simulink model "untitled1"  (R2023b)
settings: Solver=VariableStepAuto  StartTime=0.0  StopTime=20  RelTol=1e-3
settings Model: Creator=user  LastModifiedBy=user

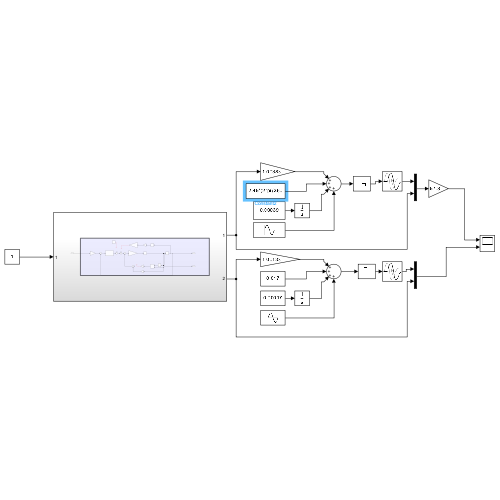
[thumbnail: Simulink's stored preview of the top-level diagram]
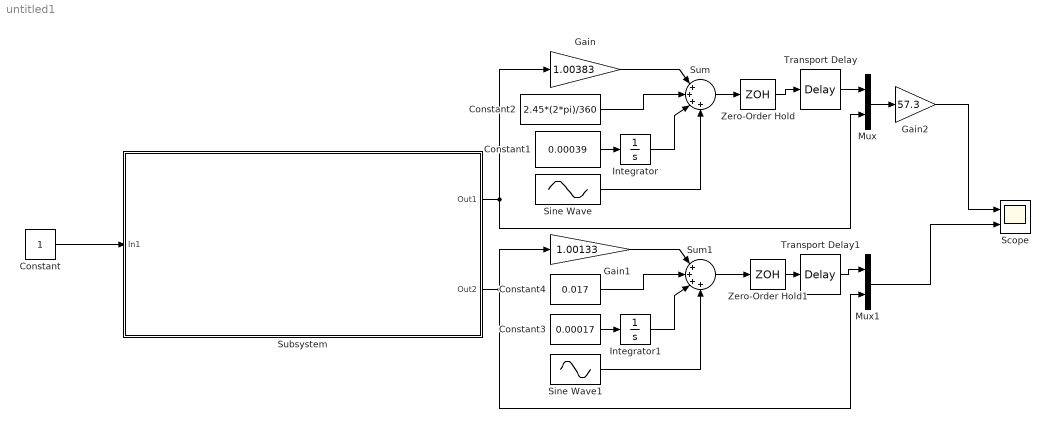
== system untitled1 ==
  Constant : Constant
  Constant1 : Constant  Value=0.00039
  Constant2 : Constant  Value=2.45*(2*pi)/360
  Constant3 : Constant  Value=0.00017
  Constant4 : Constant  Value=0.017
  Gain : Gain  Gain=1.00383
  Gain1 : Gain  Gain=1.00133
  Gain2 : Gain  Gain=57.3
  Integrator : Integrator
  Integrator1 : Integrator
  Mux : Mux  Inputs=2
  Mux1 : Mux  Inputs=2
  Scope : Scope  NumInputPorts=2
  Sine Wave : Sin  Amplitude=0.003  Frequency=50  SampleTime=0
  Sine Wave1 : Sin  Amplitude=0.00017  Frequency=25  SampleTime=0
  Subsystem : Subsystem
  Sum : Sum  Inputs=|++++
  Sum1 : Sum  Inputs=|++++
  Transport Delay : TransportDelay  DelayTime=0.002
  Transport Delay1 : TransportDelay  DelayTime=0.002
  Zero-Order Hold : ZeroOrderHold  SampleTime=0.1
  Zero-Order Hold1 : ZeroOrderHold  SampleTime=0.1
  wires:
  Constant/1 -> Subsystem/1(In1)
  Sum/1 -> Zero-Order Hold/1
  Constant1/1 -> Integrator/1
  Subsystem/1(Out1) -> Gain/1, Mux/2
  Gain/1 -> Sum/1
  Constant2/1 -> Sum/2
  Integrator/1 -> Sum/3
  Sine Wave/1 -> Sum/4
  Zero-Order Hold/1 -> Transport Delay/1
  Transport Delay1/1 -> Mux1/1
  Gain1/1 -> Sum1/1
  Zero-Order Hold1/1 -> Transport Delay1/1
  Integrator1/1 -> Sum1/3
  Sine Wave1/1 -> Sum1/4
  Subsystem/2(Out2) -> Gain1/1, Mux1/2
  Constant4/1 -> Sum1/2
  Sum1/1 -> Zero-Order Hold1/1
  Constant3/1 -> Integrator1/1
  Mux/1 -> Gain2/1
  Mux1/1 -> Scope/2
  Gain2/1 -> Scope/1
  Transport Delay/1 -> Mux/1

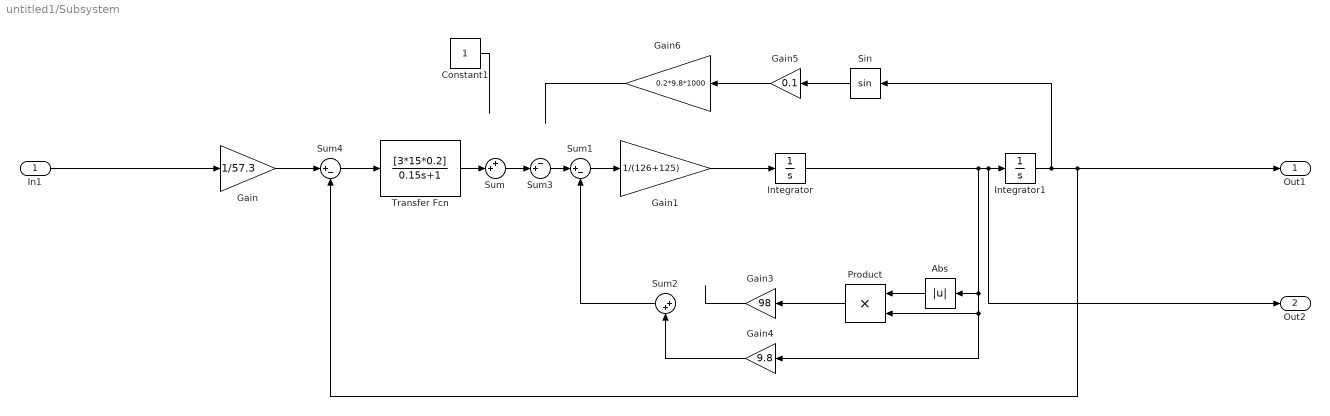
== system untitled1/Subsystem ==
  In1 : Inport
  Abs : Abs  SaturateOnIntegerOverflow=off
  Constant1 : Constant
  Gain : Gain  Gain=1/57.3
  Gain1 : Gain  Gain=1/(126+125)
  Gain3 : Gain  Gain=98
  Gain4 : Gain  Gain=9.8
  Gain5 : Gain  Gain=0.1
  Gain6 : Gain  Gain=0.2*9.8*1000
  Integrator : Integrator
  Integrator1 : Integrator
  Product : Product
  Sin : Trigonometry
  Sum : Sum  Inputs=++|
  Sum1 : Sum  Inputs=|+-
  Sum2 : Sum  Inputs=|++
  Sum3 : Sum  Inputs=-+|
  Sum4 : Sum  Inputs=|+-
  Transfer Fcn : TransferFcn  Numerator=[3*15*0.2]  Denominator=[0.15 1]
  Out1 : Outport
  Out2 : Outport  Port=2
  wires:
  Integrator/1 -> Gain4/1, Product/2, Abs/1, Out2/1, Integrator1/1
  Gain4/1 -> Sum2/2
  Sum/1 -> Sum3/2
  Sum2/1 -> Sum1/2
  Product/1 -> Gain3/1
  Sin/1 -> Gain5/1
  Sum3/1 -> Sum1/1
  Constant1/1 -> ?
  Transfer Fcn/1 -> Sum/2
  Gain6/1 -> ?
  Sum1/1 -> Gain1/1
  Gain1/1 -> Integrator/1
  Abs/1 -> Product/1
  Gain3/1 -> ?
  Gain5/1 -> Gain6/1
  In1/1 -> Gain/1
  Integrator1/1 -> Sum4/2, Out1/1, Sin/1
  Gain/1 -> Sum4/1
  Sum4/1 -> Transfer Fcn/1
